simulink model "LonLPVSim"  (R2021b)
settings: Solver=VariableStepAuto  StartTime=0.0  StopTime=10  MinStep=0.005  RelTol=1e-3
values from neighbouring files (symbols this model uses):
  LTI_lat = ss(A_lat,B_lat,C_lat,D_lat)    [Dorobantu.m]    (also in mainLinear.m = GTM_lat(:,:,i,j,k))
  s = tf('s')    [SingleDOF.m]    (also in main.m; mainSimple.m; newmain.m)
undefined symbols (not defined in the file or in its folder): ft, Hinf
libraries: simulink_extras x8, LPVBlockLibrary x4, aerolibconvert2 x1
settings Model: Creator=jihoo  LastModifiedBy=jihoo

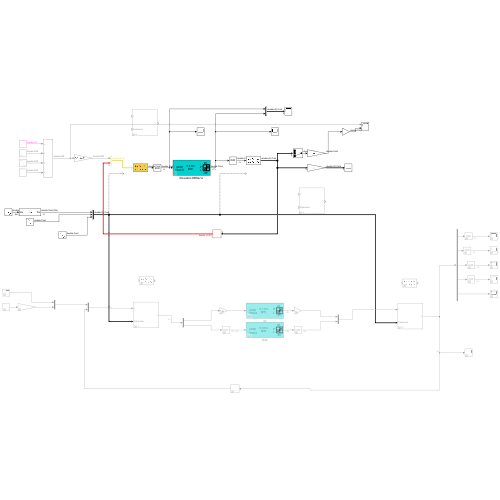
[thumbnail: Simulink's stored preview of the top-level diagram]
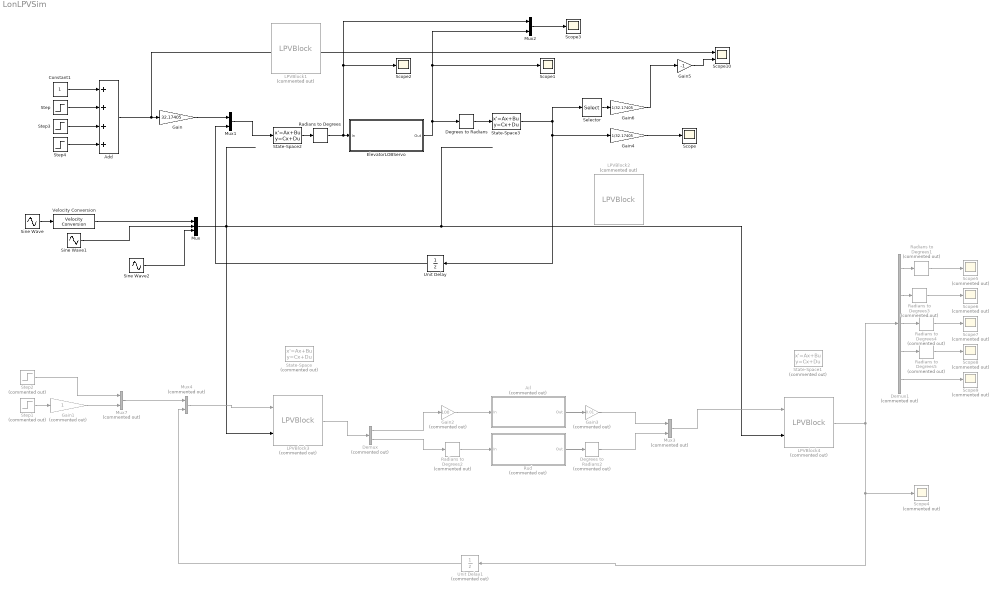
== system LonLPVSim ==
  Add : Sum  Inputs=++++
  Ail : Subsystem  Commented=on  mask(Rate and Position Limited Servo){freq=0.15, RL=300, POS_hi=25, POS_lo=-25, Bias=0}
      mask prompts: freq "Bandwidth, Hz"; RL "Rate Limit:"; POS_hi "Position Limit High:"; POS_lo "Position Limit Low:"; Bias "Bias Value:"
      mask help:
      | First order transfer function: w/(s+w), with rate and position limits
      | and output bias level.
      mask Display:
      | text(.48,.55,sprintf('%3.1f Hz\nBW',freq),'horizontalAlignment','center');
      | 
      | text(0.18,0.45,sprintf('|d/dt|\n<%0.1f',RL),'horizontalAlignment','center');
      | 
      | text(0.88,0.85,num2str(POS_hi),'horizontalAlignment', 'center');
      | text(0.88,0.2,num2str(POS_lo),'horizontalAlignment', 'center');
      | text(0.73,0.5,'P\nL');
      | 
      | 
      | plot([0.83 0.87 0.93 0.97],[0.4 0.4 0.6 0.6]);
      | plot([0.81 0.99],[0.5 0.5]);
      | plot([0.9 0.9],[0.3 0.7]);
      | plot([0.81 0.99 0.99 0.81 0.81],[0.3 0.3 0.7 0.7 0.3]);
  Constant1 : Constant
  Degrees to Radians : simulink_extras/Transformations/Degrees to Radians
  Degrees to Radians2 : simulink_extras/Transformations/Degrees to Radians  Commented=on
  Demux : Demux  Commented=on  Outputs=2
  Demux1 : Demux  Commented=on  Outputs=5
  ElevatorLOBServo : Subsystem  mask(Rate and Position Limited Servo){freq=5, RL=300, POS_hi=20, POS_lo=-30, Bias=0}
      mask prompts: freq "Bandwidth, Hz"; RL "Rate Limit:"; POS_hi "Position Limit High:"; POS_lo "Position Limit Low:"; Bias "Bias Value:"
      mask help:
      | First order transfer function: w/(s+w), with rate and position limits
      | and output bias level.
      mask Display:
      | text(.48,.55,sprintf('%3.1f Hz\nBW',freq),'horizontalAlignment','center');
      | 
      | text(0.18,0.45,sprintf('|d/dt|\n<%0.1f',RL),'horizontalAlignment','center');
      | 
      | text(0.88,0.85,num2str(POS_hi),'horizontalAlignment', 'center');
      | text(0.88,0.2,num2str(POS_lo),'horizontalAlignment', 'center');
      | text(0.73,0.5,'P\nL');
      | 
      | 
      | plot([0.83 0.87 0.93 0.97],[0.4 0.4 0.6 0.6]);
      | plot([0.81 0.99],[0.5 0.5]);
      | plot([0.9 0.9],[0.3 0.7]);
      | plot([0.81 0.99 0.99 0.81 0.81],[0.3 0.3 0.7 0.7 0.3]);
  Gain : Gain  Gain=32.17405
  Gain1 : Gain  Commented=on
  Gain2 : Gain  Commented=on  Gain=100
  Gain3 : Gain  Commented=on  Gain=0.01
  Gain4 : Gain  Gain=1/32.17405
  Gain5 : Gain  Gain=-1
  Gain6 : Gain  Gain=1/32.17405
  LPVBlock1 : LPVBlockLibrary/LPVBlock  Commented=on  sys=K_lon_hinf  plist={'rho1_tas_param';'rho2_alt_param';'rho3_mor_param'}  x0=0
      settings: SourceProductName=LPVTools Blocks
  LPVBlock2 : LPVBlockLibrary/LPVBlock  Commented=on  sys=P_lon  plist={'rho1_tas_param';'rho2_alt_param';'rho3_mor_param'}  x0=0
      settings: SourceProductName=LPVTools Blocks
  LPVBlock3 : LPVBlockLibrary/LPVBlock  Commented=on  sys=K_lat_hinf  plist={'rho1_tas_param';'rho2_alt_param';'rho3_mor_param'}  x0=0
      settings: SourceProductName=LPVTools Blocks
  LPVBlock4 : LPVBlockLibrary/LPVBlock  Commented=on  sys=P_lat  plist={'rho1_tas_param';'rho2_alt_param';'rho3_mor_param'}  x0=0
      settings: SourceProductName=LPVTools Blocks
  Mux : Mux  Inputs=3
  Mux1 : Mux  Inputs=2
  Mux2 : Mux  Inputs=2
  Mux3 : Mux  Commented=on  Inputs=2
  Mux4 : Mux  Commented=on  Inputs=2
  Mux7 : Mux  Commented=on  Inputs=2
  Radians to Degrees : simulink_extras/Transformations/Radians to Degrees
  Radians to Degrees{1..5} (5 alike) : simulink_extras/Transformations/Radians to Degrees  Commented=on
  Rud : Subsystem  Commented=on  mask(Rate and Position Limited Servo){freq=5, RL=300, POS_hi=20, POS_lo=-30, Bias=0}
      mask prompts: freq "Bandwidth, Hz"; RL "Rate Limit:"; POS_hi "Position Limit High:"; POS_lo "Position Limit Low:"; Bias "Bias Value:"
      mask help:
      | First order transfer function: w/(s+w), with rate and position limits
      | and output bias level.
      mask Display:
      | text(.48,.55,sprintf('%3.1f Hz\nBW',freq),'horizontalAlignment','center');
      | 
      | text(0.18,0.45,sprintf('|d/dt|\n<%0.1f',RL),'horizontalAlignment','center');
      | 
      | text(0.88,0.85,num2str(POS_hi),'horizontalAlignment', 'center');
      | text(0.88,0.2,num2str(POS_lo),'horizontalAlignment', 'center');
      | text(0.73,0.5,'P\nL');
      | 
      | 
      | plot([0.83 0.87 0.93 0.97],[0.4 0.4 0.6 0.6]);
      | plot([0.81 0.99],[0.5 0.5]);
      | plot([0.9 0.9],[0.3 0.7]);
      | plot([0.81 0.99 0.99 0.81 0.81],[0.3 0.3 0.7 0.7 0.3]);
  Scope{,1..3} (4 alike) : Scope
  Scope10 : Scope  NumInputPorts=2
  Scope{4..9} (6 alike) : Scope  Commented=on
  Selector : Selector  InputPortWidth=3  IndexOptions=Index vector (dialog)  Indices=3  OutputSizes=1
  Sine Wave : Sin  Amplitude=0  Bias=85  SampleTime=0
  Sine Wave1 : Sin  Amplitude=0  Bias=3000  SampleTime=0
  Sine Wave2 : Sin  Amplitude=0  Bias=-0.125  SampleTime=0
  State-Space : StateSpace  Commented=on  A=Hinf.A  B=Hinf.B  C=Hinf.C  D=Hinf.D  InitialCondition=0
  State-Space1 : StateSpace  Commented=on  A=LTI_lat.A  B=LTI_lat.B  C=LTI_lat.C  D=LTI_lat.D  InitialCondition=0
  State-Space2 : StateSpace  A=Hinf.A  B=Hinf.B  C=Hinf.C  D=Hinf.D  InitialCondition=0
  State-Space3 : StateSpace  A=LTI_lat.A  B=LTI_lat.B  C=LTI_lat.C  D=LTI_lat.D  InitialCondition=0
  Step : Step  SampleTime=0
  Step1 : Step  Commented=on  Time=3  After=10*pi/180  SampleTime=0
  Step2 : Step  Commented=on  Time=3  After=0  SampleTime=0
  Step3 : Step  Time=5  After=-2  SampleTime=0
  Step4 : Step  Time=9  SampleTime=0
  Unit Delay : UnitDelay  SampleTime=-1  HasFrameUpgradeWarning=on
  Unit Delay1 : UnitDelay  Commented=on  SampleTime=-1  HasFrameUpgradeWarning=on
  Velocity Conversion : aerolibconvert2/Velocity Conversion  IU=kts  OU=ft/s
  wires:
  State-Space2/1 -> Radians to Degrees/1
  Sine Wave/1 -> Velocity Conversion/1
  Sine Wave2/1 -> Mux/3
  Sine Wave1/1 -> Mux/2
  Mux/1 -> LPVBlock3/2, LPVBlock4/2
  Mux1/1 -> State-Space2/1
  State-Space3/1 -> Unit Delay/1, Gain4/1, Selector/1
  ElevatorLOBServo/1(Out) -> Mux2/2, Scope1/1, Degrees to Radians/1
  Velocity Conversion/1 -> Mux/1
  Add/1 -> Scope10/1, Gain/1
  Gain/1 -> Mux1/1
  Radians to Degrees/1 -> Mux2/1, Scope2/1, ElevatorLOBServo/1(In)
  Degrees to Radians/1 -> State-Space3/1
  Mux2/1 -> Scope3/1
  Demux/2 -> Radians to Degrees2/1
  Step1/1 -> Gain1/1
  Mux4/1 -> LPVBlock3/1
  Demux/1 -> Gain2/1
  Gain1/1 -> Mux7/2
  Step2/1 -> Mux7/1
  Mux7/1 -> Mux4/1
  Unit Delay/1 -> Mux1/2
  Gain4/1 -> Scope/1
  LPVBlock4/1 -> Scope4/1, Unit Delay1/1, Demux1/1
  Unit Delay1/1 -> Mux4/2
  LPVBlock3/1 -> Demux/1
  Gain2/1 -> Ail/1(In)
  Radians to Degrees2/1 -> Rud/1(In)
  Mux3/1 -> LPVBlock4/1
  Gain3/1 -> Mux3/1
  Degrees to Radians2/1 -> Mux3/2
  Demux1/1 -> Radians to Degrees1/1
  Demux1/2 -> Radians to Degrees3/1
  Demux1/3 -> Radians to Degrees4/1
  Demux1/4 -> Radians to Degrees5/1
  Demux1/5 -> Scope9/1
  Ail/1(Out) -> Gain3/1
  Rud/1(Out) -> Degrees to Radians2/1
  Radians to Degrees1/1 -> Scope5/1
  Radians to Degrees3/1 -> Scope6/1
  Radians to Degrees4/1 -> Scope7/1
  Radians to Degrees5/1 -> Scope8/1
  Gain5/1 -> Scope10/2
  Selector/1 -> Gain6/1
  Gain6/1 -> Gain5/1
  Step/1 -> Add/2
  Constant1/1 -> Add/1
  Step3/1 -> Add/3
  Step4/1 -> Add/4

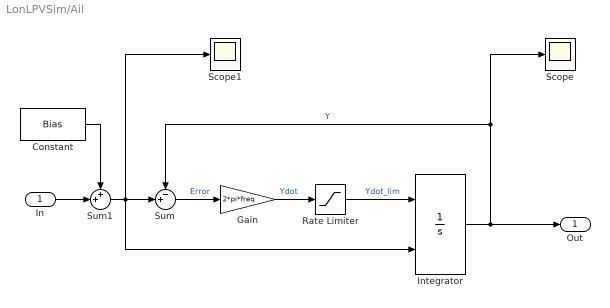
== system LonLPVSim/Ail ==
  In : Inport
  Constant : Constant  Value=Bias
  Gain : Gain  Gain=2*pi*freq  SaturateOnIntegerOverflow=on  OutDataTypeStr=Inherit: Same as input  ParamDataTypeStr=Inherit: Same as input
  Integrator : Integrator  InitialConditionSource=external  LimitOutput=on  UpperSaturationLimit=POS_hi  LowerSaturationLimit=POS_lo  IgnoreLimit=on
  Rate Limiter : Saturate  UpperLimit=RL  LowerLimit=-RL
  Scope : Scope
  Scope1 : Scope
  Sum : Sum  Inputs=-+|  InputSameDT=on  SaturateOnIntegerOverflow=on  OutDataTypeStr=Inherit: Same as first input
  Sum1 : Sum  Inputs=++|  InputSameDT=on  SaturateOnIntegerOverflow=on  OutDataTypeStr=Inherit: Same as first input
  Out : Outport  PortDimensions=1
  wires:
  Constant/1 -> Sum1/1
  Sum1/1 -> Scope1/1, Integrator/2, Sum/2
  In/1 -> Sum1/2
  Rate Limiter/1 -> Integrator/1  "Ydot_lim"
  Integrator/1 -> Out/1, Scope/1, Sum/1  "Y"
  Sum/1 -> Gain/1  "Error"
  Gain/1 -> Rate Limiter/1  "Ydot"

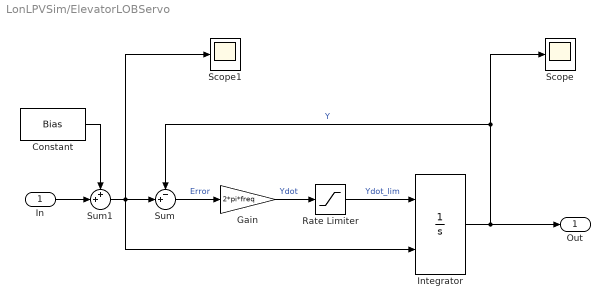
== system LonLPVSim/ElevatorLOBServo ==
  In : Inport
  Constant : Constant  Value=Bias
  Gain : Gain  Gain=2*pi*freq  SaturateOnIntegerOverflow=on  OutDataTypeStr=Inherit: Same as input  ParamDataTypeStr=Inherit: Same as input
  Integrator : Integrator  InitialConditionSource=external  LimitOutput=on  UpperSaturationLimit=POS_hi  LowerSaturationLimit=POS_lo  IgnoreLimit=on
  Rate Limiter : Saturate  UpperLimit=RL  LowerLimit=-RL
  Scope : Scope
  Scope1 : Scope
  Sum : Sum  Inputs=-+|  InputSameDT=on  SaturateOnIntegerOverflow=on  OutDataTypeStr=Inherit: Same as first input
  Sum1 : Sum  Inputs=++|  InputSameDT=on  SaturateOnIntegerOverflow=on  OutDataTypeStr=Inherit: Same as first input
  Out : Outport  PortDimensions=1
  wires:
  Constant/1 -> Sum1/1
  Sum1/1 -> Scope1/1, Integrator/2, Sum/2
  In/1 -> Sum1/2
  Rate Limiter/1 -> Integrator/1  "Ydot_lim"
  Integrator/1 -> Out/1, Scope/1, Sum/1  "Y"
  Sum/1 -> Gain/1  "Error"
  Gain/1 -> Rate Limiter/1  "Ydot"

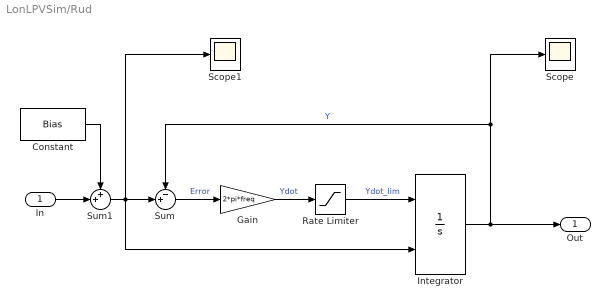
== system LonLPVSim/Rud ==
  In : Inport
  Constant : Constant  Value=Bias
  Gain : Gain  Gain=2*pi*freq  SaturateOnIntegerOverflow=on  OutDataTypeStr=Inherit: Same as input  ParamDataTypeStr=Inherit: Same as input
  Integrator : Integrator  InitialConditionSource=external  LimitOutput=on  UpperSaturationLimit=POS_hi  LowerSaturationLimit=POS_lo  IgnoreLimit=on
  Rate Limiter : Saturate  UpperLimit=RL  LowerLimit=-RL
  Scope : Scope
  Scope1 : Scope
  Sum : Sum  Inputs=-+|  InputSameDT=on  SaturateOnIntegerOverflow=on  OutDataTypeStr=Inherit: Same as first input
  Sum1 : Sum  Inputs=++|  InputSameDT=on  SaturateOnIntegerOverflow=on  OutDataTypeStr=Inherit: Same as first input
  Out : Outport  PortDimensions=1
  wires:
  Gain/1 -> Rate Limiter/1  "Ydot"
  Sum/1 -> Gain/1  "Error"
  Integrator/1 -> Sum/1, Scope/1, Out/1  "Y"
  Rate Limiter/1 -> Integrator/1  "Ydot_lim"
  In/1 -> Sum1/2
  Sum1/1 -> Sum/2, Integrator/2, Scope1/1
  Constant/1 -> Sum1/1
